simulink model "XAUTO01_reference"  (R2025a)
settings: Solver=FixedStepDiscrete  StartTime=0  StopTime=9.5  FixedStep=0.002  RelTol=1e-3
undefined symbols (not defined in the file): brake_demand, brake_onset, friction_drop, friction_event_time, initial_speed, left_friction, right_friction, vehicle_mass
settings Model: Creator=SimuVerity Contributors  LastModifiedBy=SimuVerity Contributors

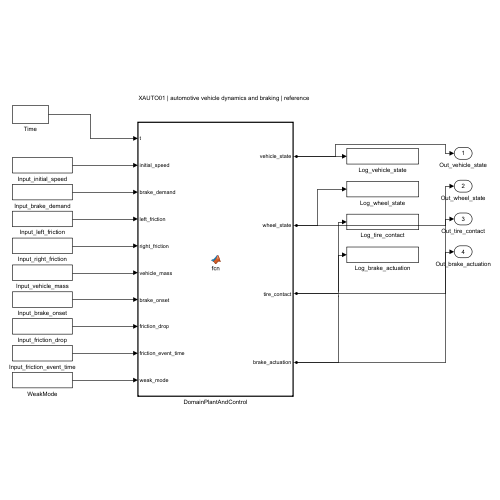
[thumbnail: Simulink's stored preview of the top-level diagram]
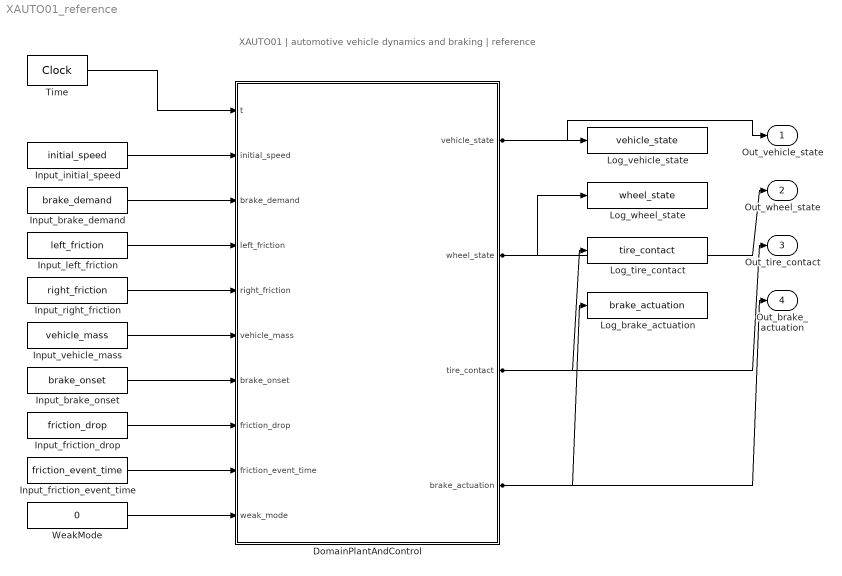
== system XAUTO01_reference ==
  note: XAUTO01 | automotive vehicle dynamics and braking | reference
  DomainPlantAndControl : MATLAB Function  TreatAsAtomicUnit=on
  Input_brake_demand : Constant  Value=brake_demand
  Input_brake_onset : Constant  Value=brake_onset
  Input_friction_drop : Constant  Value=friction_drop
  Input_friction_event_time : Constant  Value=friction_event_time
  Input_initial_speed : Constant  Value=initial_speed
  Input_left_friction : Constant  Value=left_friction
  Input_right_friction : Constant  Value=right_friction
  Input_vehicle_mass : Constant  Value=vehicle_mass
  Log_brake_actuation : ToWorkspace  VariableName=brake_actuation  SaveFormat=Timeseries  SampleTime=-1
  Log_tire_contact : ToWorkspace  VariableName=tire_contact  SaveFormat=Timeseries  SampleTime=-1
  Log_vehicle_state : ToWorkspace  VariableName=vehicle_state  SaveFormat=Timeseries  SampleTime=-1
  Log_wheel_state : ToWorkspace  VariableName=wheel_state  SaveFormat=Timeseries  SampleTime=-1
  Time : DigitalClock  SampleTime=0.002
  WeakMode : Constant  Value=0
  Out_vehicle_state : Outport
  Out_wheel_state : Outport  Port=2
  Out_tire_contact : Outport  Port=3
  Out_brake_actuation : Outport  Port=4
  wires:
  Time/1 -> DomainPlantAndControl/1(t)
  Input_initial_speed/1 -> DomainPlantAndControl/2(initial_speed)
  Input_brake_demand/1 -> DomainPlantAndControl/3(brake_demand)
  Input_left_friction/1 -> DomainPlantAndControl/4(left_friction)
  Input_right_friction/1 -> DomainPlantAndControl/5(right_friction)
  Input_vehicle_mass/1 -> DomainPlantAndControl/6(vehicle_mass)
  Input_brake_onset/1 -> DomainPlantAndControl/7(brake_onset)
  Input_friction_drop/1 -> DomainPlantAndControl/8(friction_drop)
  Input_friction_event_time/1 -> DomainPlantAndControl/9(friction_event_time)
  WeakMode/1 -> DomainPlantAndControl/10(weak_mode)
  DomainPlantAndControl/1(vehicle_state) -> Log_vehicle_state/1, Out_vehicle_state/1
  DomainPlantAndControl/2(wheel_state) -> Log_wheel_state/1, Out_wheel_state/1
  DomainPlantAndControl/3(tire_contact) -> Log_tire_contact/1, Out_tire_contact/1
  DomainPlantAndControl/4(brake_actuation) -> Log_brake_actuation/1, Out_brake_actuation/1

== matlab function XAUTO01_reference/DomainPlantAndControl ==
  data: t input; vehicle_state output; initial_speed input; brake_demand input; left_friction input; right_friction input; vehicle_mass input; brake_onset input; friction_drop input; friction_event_time input; weak_mode input; wheel_state output; tire_contact output; brake_actuation output
function [vehicle_state,wheel_state,tire_contact,brake_actuation] = fcn(t,initial_speed,brake_demand,left_friction,right_friction,vehicle_mass,brake_onset,friction_drop,friction_event_time,weak_mode)
%#codegen
persistent x y psi vx yawRate omega torque integ
dt=0.002; g=9.81; Rt=0.31; track=1.62; Jw=1.85; m=vehicle_mass; Izz=1.65*m;
if isempty(x) || t<0.5*dt
    x=0; y=0; psi=0; vx=initial_speed; yawRate=0;
    omega=(initial_speed/Rt)*ones(1,4); torque=zeros(1,4); integ=zeros(1,4);
end
active=double(t>=brake_onset); event=double(t>=friction_event_time && t<friction_event_time+1.0);
Fz=[0.285*m*g,0.285*m*g,0.215*m*g,0.215*m*g];
mu=[left_friction,right_friction*(1-friction_drop*event),left_friction,right_friction*(1-friction_drop*event)];
vWheel=[vx-0.5*track*yawRate,vx+0.5*track*yawRate,vx-0.5*track*yawRate,vx+0.5*track*yawRate];
slip=(vWheel-Rt*omega)./max(abs(vWheel),0.55); slip=min(max(slip,-0.35),1.25);
Fx=mu.*Fz.*tanh(slip/0.115);
if weak_mode<0.5
    targetSlip=.06+.11*brake_demand; e=targetSlip-slip; integ=min(max(integ+active*e*dt,-0.35),0.35);
    feed=Rt*mu.*Fz.*tanh(targetSlip/.115); desired=active*(feed+5600*e+1350*integ);
    stability=min(max(35000*(psi+0.22*yawRate),-2800),2800);
    desired([1 3])=desired([1 3])-stability; desired([2 4])=desired([2 4])+stability;
    desired=min(max(desired,0),4600*brake_demand);
else
    desired=(4050*brake_demand*active)*ones(1,4);
end
torque=torque+dt*(desired-torque)/0.028;
domega=(Rt*Fx-torque-0.02*omega)/Jw; omega=max(omega+dt*domega,0);
drag=0.42*vx*abs(vx); dv=-(sum(Fx)+drag)/m;
Mz=((Fx(1)+Fx(3))-(Fx(2)+Fx(4)))*0.5*track-6500*yawRate-75000*psi;
dyaw=Mz/Izz; vx=max(vx+dt*dv,0); yawRate=yawRate+dt*dyaw;
if vx<0.08, vx=0; omega(:)=0; torque=0.92*torque; yawRate=0.96*yawRate; end
psi=psi+dt*yawRate; x=x+dt*vx*cos(psi); y=y+dt*vx*sin(psi);
vWheel=[vx-0.5*track*yawRate,vx+0.5*track*yawRate,vx-0.5*track*yawRate,vx+0.5*track*yawRate];
slip=(vWheel-Rt*omega)./max(abs(vWheel),0.55); slip=min(max(slip,-0.35),1.25);
vehicle_state=[x,y,psi,vx,yawRate];
wheel_state=[omega,slip];
tire_contact=[Fx,Fz,mu(1),mu(2)];
brake_actuation=[torque,brake_demand*active];
end
